simulink model "ex5_8"  (R2026a)
settings: Solver=FixedStepAuto  StopTime=5  FixedStep=0.001
settings Model: Creator=User  LastModifiedBy=User

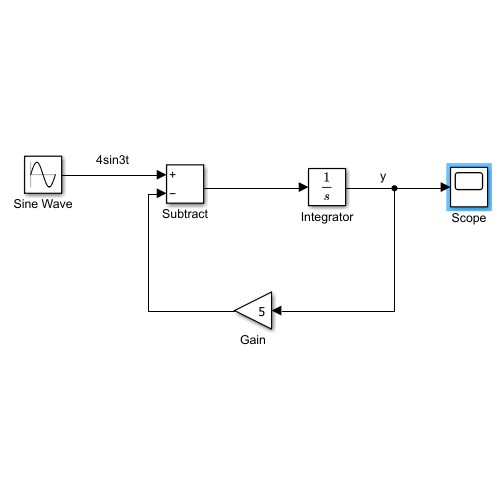
[thumbnail: Simulink's stored preview of the top-level diagram]
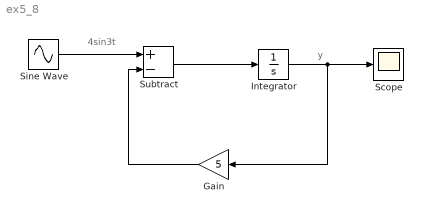
== system ex5_8 ==
  note: y
  note: 4sin3t
  Gain : Gain  Gain=5
  Integrator : Integrator  InitialCondition=1
  Scope : Scope
      settings: ActiveDisplayYMinimum=-1.0080836027333151  ActiveDisplayYMaximum=1.3151333507958827
  Sine Wave : Sin  Amplitude=4  Frequency=3  SampleTime=0
  Subtract : Sum  Inputs=+-
  wires:
  Sine Wave/1 -> Subtract/1
  Subtract/1 -> Integrator/1
  Integrator/1 -> Gain/1, Scope/1
  Gain/1 -> Subtract/2
